simulink library "sm_robot_run_4legs_lib"  (R2025a)
settings: Solver=ode45  StartTime=0.0  StopTime=10.0  RelTol=1e-3
values from neighbouring files (symbols this model uses):
  N = 100    [Extr_Data_Cam_Roller_Curve.m]
  s = sin(q)    [Extr_Data_Cam_Roller_Curve.m]
undefined symbols (not defined in the file or in its folder): bw, d2r, Extr_Data_LinkEndHole, ground, J, joint_damping, k2, knee_torque, l1, l2, L_back, m1, m2, r2d, T_cg, t_th, t_w, th2, Trq_propulsive, u_th, u_w, X, Y, Z
libraries: sm_lib x25, nesl_utility x14, fl_lib x13, Contact_Forces_Lib x1, ee_lib x1
(part 1 of 2)
Description:
  | Copyright 2012-2025 The MathWorks, Inc.
settings Model: Creator=rhyde  LastModifiedBy=smiller
settings SolverCC: AlgebraicLoopSolver=TrustRegion
settings DataIOCC: SaveFormat=Array  SignalLoggingSaveFormat=ModelDataLogs  ReturnWorkspaceOutputs=off
settings OptimizationCC: BlockReduction=off  BooleanDataType=off  ReuseModelBlockBuffer=off  ExpressionDepthLimit=2147483647.0  LifeSpan=inf
settings DebuggingCC: SaveWithParameterizedLinksMsg=none  UnderspecifiedInitializationDetection=Classic  MergeDetectMultiDrivingBlocksExec=none  SignalResolutionControl=TryResolveAllWithWarning  UnconnectedInputMsg=warning  UnconnectedOutputMsg=warning  UnconnectedLineMsg=warning  StateNameClashWarn=warning  PregeneratedLibrarySubsystemCodeDiagnostic=none  SFUnexpectedBacktrackingDiag=warning  SFNoUnconditionalDefaultTransitionDiag=warning  SFExecutionAtInitializationDiag=none  ArithmeticOperatorsInVariantConditions=warning
settings HardwareCC: ProdBitPerPointer=32.0  ProdBitPerSizeT=32.0  ProdBitPerPtrDiffT=32.0  ProdLargestAtomicFloat=None  ProdIntDivRoundTo=Undefined  ProdEndianess=Unspecified  ProdWordSize=32.0  ProdHWDeviceType=32-bit Generic  TargetUnknown=on
settings ModelReferenceCC: EnableRefExpFcnMdlSchedulingChecks=on  PropagateSignalLabelsOutOfModel=off
settings SFSimCC: SimUseLocalCustomCode=off  CustomCodeUndefinedFunction=UseInterfaceOnly
settings RTWCC: RTWUseLocalCustomCode=off  GPUComputeCapability=3.5  DLArmComputeVersion=19.05
settings CodeAppCC: StateflowObjectComments=on
settings GRTTargetCC: TargetLangStandard=C89/C90 (ANSI)
settings ConfigComp: CovMetricSettings=dw  CovSaveCumulativeToWorkspaceVar=on  CovSaveSingleToWorkspaceVar=on  CovExternalEMLEnable=off

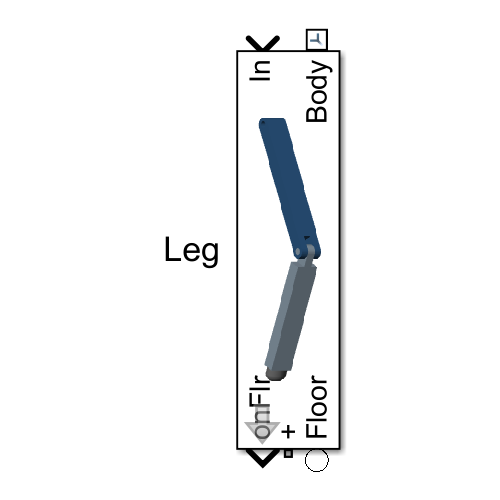
[thumbnail: Simulink's stored preview of the top-level diagram]
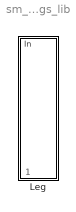
== system sm_robot_run_4legs_lib ==
  Leg : Subsystem  Tag=PublishSubsystemCustomStyle  mask{leg_type=Front Left, leg_width=0.1*l1, th1_0=d2r*u_th(find(t_th > 3*T_cg/4,1)), th2_0=-50*d2r+th2, th1_dot_0=-d2r*u_w(find(t_th > 3*T_cg/4,1)), x0=L_back, popup_contact_model=Planar}
      mask prompts: leg_type "Leg type"; leg_width "Leg width (m)"; th1_0 "Initial hip angle, th1_0"; th2_0 "Initial knee angle, th2_0"; th1_dot_0 "Initial hip angular velocity"; x0 "Current or last ground contact position, x0"; popup_contact_model "Contact Force Model"
      mask init:
      | if (leg_type == 1 || leg_type == 3)
      |     sideSign = -1;
      | else
      |     sideSign = 1;
      | end
      | 
      | if (popup_contact_model==1)
      |     set_param([gcb '/Contact Force Model'],'OverrideUsingVariant','Planar');
      | else
      |     set_param([gcb '/Contact Force Model'],'OverrideUsingVariant','SixDOF');
      | end
      mask TypeOptions leg_type: Front Left | Front Right | Rear Left | Rear Right
      mask TypeOptions popup_contact_model: Planar | Six DOF
      mask Display: image('sm_robot_run_leg_IMAGE.png')

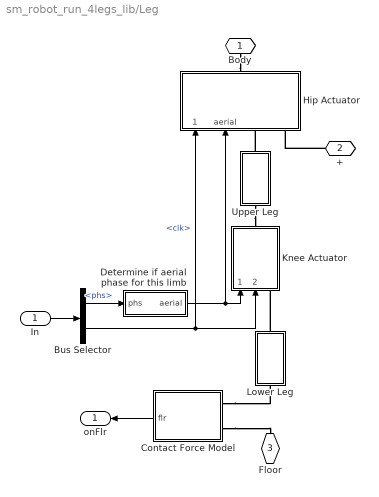
== system sm_robot_run_4legs_lib/Leg ==
  In : Inport
  Bus Selector : BusSelector  OutputSignals=phs,clk
  Contact Force Model : Subsystem  Variant=on  VariantControlMode=label  VariantControl=ThreeDim  LabelModeActiveChoice=Planar
      settings: AttributesFormatString=%<ActiveVariant>
      mask Display: disp(' ');
  Determine if aerial phase for this limb : Subsystem
  Hip Actuator : Subsystem
  Knee Actuator : Subsystem
  Lower Leg : Subsystem
  Upper Leg : Subsystem
  Body : PMIOPort  Side=Left
  + : PMIOPort  Port=2  Side=Right
  Floor : PMIOPort  Tag=PMCPort  Port=3  Side=Right
  onFlr : Outport  VectorParamsAs1DForOutWhenUnconnected=off
  wires:
  Contact Force Model/1("  flr") -> onFlr/1
  Bus Selector/2 -> Knee Actuator/2(t_aerial), Hip Actuator/1(t_aerial)  "<clk>"
  Determine if aerial phase for this limb/1(aerial) -> Knee Actuator/1(aerial), Hip Actuator/2(aerial)
  In/1 -> Bus Selector/1
  Bus Selector/1 -> Determine if aerial phase for this limb/1(phs)  "<phs>"
  connections:
  Body/RConn1 -- Hip Actuator/RConn1
  +/RConn1 -- Hip Actuator/LConn2
  Lower Leg/RConn1 -- Knee Actuator/LConn1
  Contact Force Model/LConn1 -- Lower Leg/LConn1
  Upper Leg/RConn1 -- Hip Actuator/LConn1
  Upper Leg/LConn1 -- Knee Actuator/RConn1
  Contact Force Model/LConn2 -- Floor/RConn1

== system sm_robot_run_4legs_lib/Leg/Contact Force Model ==
  Planar : Subsystem  VariantControl=Planar
  SixDOF : Subsystem  VariantControl=SixDOF
  " F " : PMIOPort  Side=Left
  " W " : PMIOPort  Port=2  Side=Left
  "  flr" : Outport  VectorParamsAs1DForOutWhenUnconnected=off

== system sm_robot_run_4legs_lib/Leg/Determine if aerial phase for this limb ==
  phs : Inport
  Aerial : Switch  Threshold=0.5  SaturateOnIntegerOverflow=off  InputSameDT=off
  "Front left or rear right leg airborne if phase is 1, 2, 3, 6, 7 or 8" : Fcn  Expr=(u(1)==1)+(u(1)==2)+(u(1)==3)+(u(1)==6)+(u(1)==7)+(u(1)==8)
  "Front right or rear left leg airborne if phase is 2, 3, 4, 5, 6 or 7" : Fcn  Expr=(u(1)==2)+(u(1)==3)+(u(1)==4)+(u(1)==5)+(u(1)==6)+(u(1)==7)
  Leg type is front right or rear left : Constant  Value=(leg_type==2)+(leg_type==3)
  aerial : Outport  VectorParamsAs1DForOutWhenUnconnected=off
  wires:
  Leg type is front right or rear left/1 -> Aerial/2
  "Front right or rear left leg airborne if phase is 2, 3, 4, 5, 6 or 7"/1 -> Aerial/1
  phs/1 -> "Front right or rear left leg airborne if phase is 2, 3, 4, 5, 6 or 7"/1, "Front left or rear right leg airborne if phase is 1, 2, 3, 6, 7 or 8"/1
  "Front left or rear right leg airborne if phase is 1, 2, 3, 6, 7 or 8"/1 -> Aerial/3
  Aerial/1 -> aerial/1

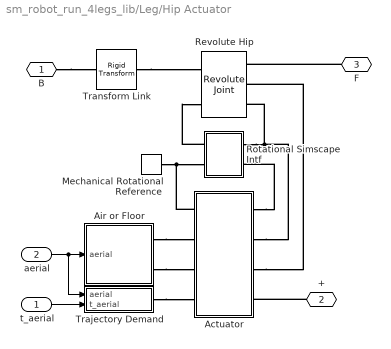
== system sm_robot_run_4legs_lib/Leg/Hip Actuator ==
  t_aerial : Inport
  aerial : Inport  Port=2
  Actuator : Subsystem
  Air or Floor : Subsystem
  Mechanical Rotational Reference : fl_lib/Mechanical/Rotational Elements/Mechanical Rotational Reference
  Revolute Hip : sm_lib/Joints/Revolute Joint  JointMode=Normal  CompositeWrenchDir=FollowerOnBase  CompositeWrenchFrame=BaseFrame  SenseConstraintForce=off  SenseConstraintTorque=off  SenseTotalForce=off  SenseTotalTorque=off  PositionTargetSpecify=on  PositionTargetPriority=High  PositionTargetValue=-th1_0  PositionTargetValueUnits=rad  VelocityTargetSpecify=on  VelocityTargetPriority=High  VelocityTargetValue=th1_dot_0  VelocityTargetValueUnits=rad/s  EquilibriumPosition=0  EquilibriumPositionUnits=deg  SpringStiffness=0  SpringStiffnessUnits=N*m/deg  DampingCoefficient=0  DampingCoefficientUnits=N*m/(deg/s)  LowerLimitSpecify=off  LowerLimitBound=-90  LowerLimitBoundUnits=deg  LowerLimitStiffness=1e4  LowerLimitStiffnessUnits=N*m/deg  LowerLimitDamping=10  LowerLimitDampingUnits=N*m/(deg/s)  LowerLimitTransitionRegionWidth=0.1  LowerLimitTransitionRegionWidthUnits=deg  UpperLimitSpecify=off  UpperLimitBound=90  UpperLimitBoundUnits=deg  UpperLimitStiffness=1e4  UpperLimitStiffnessUnits=N*m/deg  UpperLimitDamping=10  UpperLimitDampingUnits=N*m/(deg/s)  UpperLimitTransitionRegionWidth=0.1  UpperLimitTransitionRegionWidthUnits=deg  TorqueActuationMode=InputTorque  MotionActuationMode=ComputedMotion  SensePosition=on  SenseVelocity=on  SenseAcceleration=off  SenseTorqueForce=off  SenseLowerLimitTorqueForce=off  SenseUpperLimitTorqueForce=off
  Rotational Simscape Intf : Subsystem
  Trajectory Demand : Subsystem
  Transform Link : sm_lib/Frames and Transforms/Rigid Transform  RotationMethod=None  FollAlignAxisA=+X  BaseAlignAxisA=+Y  FollAlignAxisB=+Y  BaseAlignAxisB=+Z  RotationStandardAxis=+Z  RotationAngle=0.0  RotationAngleUnits=deg  RotationArbitraryAxis=[0 0 1]  RotationSequenceAxes=FollowerAxes  RotationSequence=XYX  RotationSequenceAngles=[0 0 0]  RotationSequenceAnglesUnits=deg  RotationMatrix=[1 0 0; 0 1 0; 0 0 1]  Quaternion=[1 0 0 0]  TranslationMethod=StandardAxis  TranslationCartesianOffset=[0 0 0]  TranslationCartesianOffsetUnits=m  TranslationStandardAxis=+Z  TranslationStandardOffset=leg_width*sideSign/2  TranslationStandardOffsetUnits=m  TranslationROffset=0  TranslationROffsetUnits=m  TranslationThetaOffset=0  TranslationThetaOffsetUnits=deg  TranslationZOffset=0  TranslationZOffsetUnits=m
  B : PMIOPort  Side=Left
  + : PMIOPort  Port=2  Side=Left
  F : PMIOPort  Port=3  Side=Right
  wires:
  aerial/1 -> Trajectory Demand/1(aerial), Air or Floor/1(aerial)
  t_aerial/1 -> Trajectory Demand/2(t_aerial)
  connections:
  Trajectory Demand/RConn1 -- Actuator/LConn4
  Mechanical Rotational Reference/LConn1 -- Actuator/LConn1 -- Rotational Simscape Intf/LConn2
  +/RConn1 -- Actuator/RConn4
  Transform Link/RConn1 -- Revolute Hip/LConn1
  F/RConn1 -- Revolute Hip/RConn1
  Actuator/RConn3 -- Revolute Hip/RConn2
  Rotational Simscape Intf/RConn1 -- Actuator/RConn2 -- Revolute Hip/RConn3
  Rotational Simscape Intf/LConn1 -- Revolute Hip/LConn2
  B/RConn1 -- Transform Link/LConn1
  Actuator/RConn1 -- Rotational Simscape Intf/RConn2
  Air or Floor/RConn2 -- Actuator/LConn3
  Air or Floor/RConn1 -- Actuator/LConn2

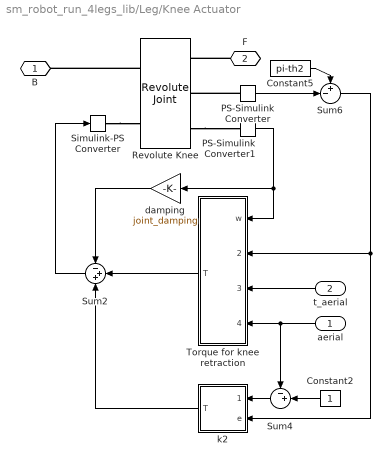
== system sm_robot_run_4legs_lib/Leg/Knee Actuator ==
  aerial : Inport
  t_aerial : Inport  Port=2
  Constant2 : Constant
  Constant5 : Constant  Value=pi-th2
  PS-Simulink Converter : nesl_utility/PS-Simulink Converter  PhysicalDomain=network_engine_domain  SubClassName=ps_output  LeftPortType=input  RightPortType=output  PseudoPeriodic=off  Frequencies=[]  VectorFormat=1-D array  Unit=rad  AffineConversion=off
  PS-Simulink Converter1 : nesl_utility/PS-Simulink Converter  PhysicalDomain=network_engine_domain  SubClassName=ps_output  LeftPortType=input  RightPortType=output  PseudoPeriodic=off  Frequencies=[]  VectorFormat=1-D array  Unit=rad/s  AffineConversion=off
  Revolute Knee : sm_lib/Joints/Revolute Joint  JointMode=Normal  CompositeWrenchDir=FollowerOnBase  CompositeWrenchFrame=BaseFrame  SenseConstraintForce=off  SenseConstraintTorque=off  SenseTotalForce=off  SenseTotalTorque=off  PositionTargetSpecify=on  PositionTargetPriority=High  PositionTargetValue=-th2_0+pi  PositionTargetValueUnits=rad  VelocityTargetSpecify=on  VelocityTargetPriority=High  VelocityTargetValue=0  VelocityTargetValueUnits=rad/s  EquilibriumPosition=0  EquilibriumPositionUnits=deg  SpringStiffness=0  SpringStiffnessUnits=N*m/deg  DampingCoefficient=0  DampingCoefficientUnits=N*m/(deg/s)  LowerLimitSpecify=off  LowerLimitBound=-90  LowerLimitBoundUnits=deg  LowerLimitStiffness=1e4  LowerLimitStiffnessUnits=N*m/deg  LowerLimitDamping=10  LowerLimitDampingUnits=N*m/(deg/s)  LowerLimitTransitionRegionWidth=0.1  LowerLimitTransitionRegionWidthUnits=deg  UpperLimitSpecify=off  UpperLimitBound=90  UpperLimitBoundUnits=deg  UpperLimitStiffness=1e4  UpperLimitStiffnessUnits=N*m/deg  UpperLimitDamping=10  UpperLimitDampingUnits=N*m/(deg/s)  UpperLimitTransitionRegionWidth=0.1  UpperLimitTransitionRegionWidthUnits=deg  TorqueActuationMode=InputTorque  MotionActuationMode=ComputedMotion  SensePosition=on  SenseVelocity=on  SenseAcceleration=off  SenseTorqueForce=off  SenseLowerLimitTorqueForce=off  SenseUpperLimitTorqueForce=off
  Simulink-PS Converter : nesl_utility/Simulink-PS Converter  PhysicalDomain=network_engine_domain  SubClassName=ps_input  LeftPortType=input  RightPortType=output  PseudoPeriodic=off  Frequencies=[]  NoiseDistribution=none  NoiseParameters=[]  Unit=1  AffineConversion=off  FilteringAndDerivatives=provide  SimscapeFilterOrder=1  InputFilterTimeConstant=0.005  UdotUserProvided=0
  Sum2 : Sum  Inputs=-++  InputSameDT=on  SaturateOnIntegerOverflow=on  OutDataTypeStr=Inherit: Same as first input
  Sum4 : Sum  Inputs=-+|  InputSameDT=on  SaturateOnIntegerOverflow=on  OutDataTypeStr=Inherit: Same as first input
  Sum6 : Sum  Inputs=+-|  InputSameDT=on  SaturateOnIntegerOverflow=on  OutDataTypeStr=Inherit: Same as first input
  Torque for knee retraction : Subsystem
  damping : Gain  Gain=joint_damping  SaturateOnIntegerOverflow=on  OutDataTypeStr=Inherit: Same as input  ParamDataTypeStr=Inherit: Same as input
  k2 : Subsystem
  B : PMIOPort  Side=Left
  F : PMIOPort  Port=2  Side=Right
  wires:
  Torque for knee retraction/1(T) -> Sum2/2
  k2/1(T) -> Sum2/3
  Constant2/1 -> Sum4/2
  Sum4/1 -> k2/1(Enable)
  aerial/1 -> Sum4/1, Torque for knee retraction/4(Enable)
  Sum6/1 -> k2/2(e), Torque for knee retraction/2(angle)
  damping/1 -> Sum2/1
  PS-Simulink Converter1/1 -> Torque for knee retraction/1(w), damping/1
  Sum2/1 -> Simulink-PS Converter/1
  t_aerial/1 -> Torque for knee retraction/3(t_aerial)
  PS-Simulink Converter/1 -> Sum6/2
  Constant5/1 -> Sum6/1
  connections:
  F/RConn1 -- Revolute Knee/RConn1
  PS-Simulink Converter/LConn1 -- Revolute Knee/RConn2
  Revolute Knee/RConn3 -- PS-Simulink Converter1/LConn1
  Simulink-PS Converter/RConn1 -- Revolute Knee/LConn2
  Revolute Knee/LConn1 -- B/RConn1

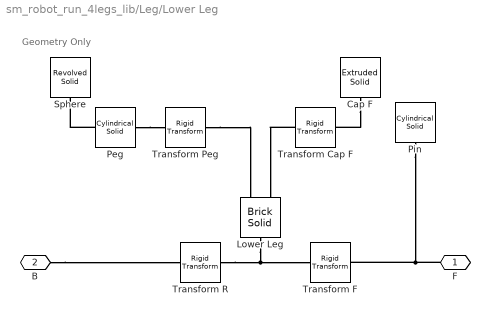
== system sm_robot_run_4legs_lib/Leg/Lower Leg ==
  note: Geometry Only
  Cap F : sm_lib/Body Elements/Extruded Solid  ExtrusionType=General  PolygonNumSides=3  PolygonOuterRadius=1  PolygonOuterRadiusUnits=m  ExportEntireGeometry=off  ExtrusionCrossSection=Extr_Data_LinkEndHole(l2*0.1,l1*0.025,0.05*l2)  ExtrusionCrossSectionUnits=m  ExportConvexHullGeometry=off  ExtrusionLength=l2*0.1/3  ExtrusionLengthUnits=m  InertiaType=CalculateFromGeometry  BasedOnType=Density  Density=0  DensityUnits=kg/m^3  Mass=1  MassUnits=kg  CenterOfMass=[0 0 0]  CenterOfMassUnits=m  MomentsOfInertia=[1 1 1]  MomentsOfInertiaUnits=kg*m^2  ProductsOfInertia=[1 1 1]  ProductsOfInertiaUnits=kg*m^2  GraphicType=FromGeometry  MarkerShape=Sphere  MarkerSize=10  GraphicVisPropType=SimpleVisualProperties  GraphicDiffuseColor=[164 184 200]/255  GraphicOpacity=1.0  GraphicSpecularColor=[0.5 0.5 0.5 1.0]  GraphicAmbientColor=[0.15 0.15 0.15 1.0]  GraphicEmissiveColor=[0.0 0.0 0.0 1.0]  GraphicShininess=75  DoExposeReferenceFrame=on  SerializedFrames=<Frames/>
  Lower Leg : sm_lib/Body Elements/Brick Solid  BrickDimensions=[0.1 0.8 0.1]*l2  BrickDimensionsUnits=m  ExportEntireGeometry=off  InertiaType=Custom  BasedOnType=Density  Density=1000  DensityUnits=kg/m^3  Mass=m2*l2  MassUnits=kg  CenterOfMass=[0 0 0]  CenterOfMassUnits=m  MomentsOfInertia=[1 1 1]*(1/12)*m2*l2*l2^2  MomentsOfInertiaUnits=kg*m^2  ProductsOfInertia=[1 1 1]*0  ProductsOfInertiaUnits=kg*m^2  GraphicType=FromGeometry  MarkerShape=Sphere  MarkerSize=10  GraphicVisPropType=SimpleVisualProperties  GraphicDiffuseColor=[164 184 200]/255  GraphicOpacity=1.0  GraphicSpecularColor=[0.5 0.5 0.5 1.0]  GraphicAmbientColor=[0.15 0.15 0.15 1.0]  GraphicEmissiveColor=[0.0 0.0 0.0 1.0]  GraphicShininess=75  DoExposeReferenceFrame=on  SerializedFrames=<Frames><Frame><Id>Frame1</Id><Value><Name>B</Name><Origin><Source>GeometricFeature</Source><FeatureName>-y surface</FeatureName></Origin><PrimaryAxis><DefinedDirection>+Z</DefinedDirection><Source>ReferenceFrame</Source><SourceDirection>+Z</SourceDirection><FeatureName></FeatureName></PrimaryAxis><SecondaryAxis><DefinedDirection>+X</DefinedDirection><Source>ReferenceFrame</Source><SourceDirection>+X</SourceDirection><FeatureName></FeatureName></SecondaryAxis></Value></Frame><Frame><Id>Frame2</Id><Value><Name>F</Name><Origin><Source>GeometricFeature</Source><FeatureName>+y surface</FeatureName></Origin><PrimaryAxis><DefinedDirection>+Z</DefinedDirection><Source>ReferenceFrame</Source><SourceDirection>+Z</SourceDirection><FeatureName></FeatureName></PrimaryAxis><SecondaryAxis><DefinedDirection>+X</DefinedDirection><Source>ReferenceFrame</Source><SourceDirection>+X</SourceDirection><FeatureName></FeatureName></SecondaryAxis></Value></Frame></Frames>
  Peg : sm_lib/Body Elements/Cylindrical Solid  CylinderRadius=0.05*l1  CylinderRadiusUnits=m  CylinderLength=0.05*l2  CylinderLengthUnits=m  ExportEntireGeometry=off  InertiaType=CalculateFromGeometry  BasedOnType=Density  Density=0  DensityUnits=kg/m^3  Mass=1  MassUnits=kg  CenterOfMass=[0 0 0]  CenterOfMassUnits=m  MomentsOfInertia=[1 1 1]  MomentsOfInertiaUnits=kg*m^2  ProductsOfInertia=[1 1 1]  ProductsOfInertiaUnits=kg*m^2  GraphicType=FromGeometry  MarkerShape=Sphere  MarkerSize=10  GraphicVisPropType=SimpleVisualProperties  GraphicDiffuseColor=[0.5 0.5 0.5]  GraphicOpacity=1.0  GraphicSpecularColor=[0.5 0.5 0.5 1.0]  GraphicAmbientColor=[0.15 0.15 0.15 1.0]  GraphicEmissiveColor=[0.0 0.0 0.0 1.0]  GraphicShininess=75  DoExposeReferenceFrame=off  SerializedFrames=<Frames><Frame><Id>Frame1</Id><Value><Name>B</Name><Origin><Source>GeometricFeature</Source><FeatureName>bottom surface</FeatureName></Origin><PrimaryAxis><DefinedDirection>+Z</DefinedDirection><Source>ReferenceFrame</Source><SourceDirection>+Z</SourceDirection><FeatureName></FeatureName></PrimaryAxis><SecondaryAxis><DefinedDirection>+X</DefinedDirection><Source>ReferenceFrame</Source><SourceDirection>+X</SourceDirection><FeatureName></FeatureName></SecondaryAxis></Value></Frame><Frame><Id>Frame2</Id><Value><Name>F</Name><Origin><Source>GeometricFeature</Source><FeatureName>top surface</FeatureName></Origin><PrimaryAxis><DefinedDirection>+Z</DefinedDirection><Source>ReferenceFrame</Source><SourceDirection>+Z</SourceDirection><FeatureName></FeatureName></PrimaryAxis><SecondaryAxis><DefinedDirection>+X</DefinedDirection><Source>ReferenceFrame</Source><SourceDirection>+X</SourceDirection><FeatureName></FeatureName></SecondaryAxis></Value></Frame></Frames>
  Pin : sm_lib/Body Elements/Cylindrical Solid  CylinderRadius=0.025*l1  CylinderRadiusUnits=m  CylinderLength=0.1*l2  CylinderLengthUnits=m  ExportEntireGeometry=off  InertiaType=CalculateFromGeometry  BasedOnType=Density  Density=0  DensityUnits=kg/m^3  Mass=1  MassUnits=kg  CenterOfMass=[0 0 0]  CenterOfMassUnits=m  MomentsOfInertia=[1 1 1]  MomentsOfInertiaUnits=kg*m^2  ProductsOfInertia=[1 1 1]  ProductsOfInertiaUnits=kg*m^2  GraphicType=FromGeometry  MarkerShape=Sphere  MarkerSize=10  GraphicVisPropType=SimpleVisualProperties  GraphicDiffuseColor=[164 184 200]/255  GraphicOpacity=1.0  GraphicSpecularColor=[0.5 0.5 0.5 1.0]  GraphicAmbientColor=[0.15 0.15 0.15 1.0]  GraphicEmissiveColor=[0.0 0.0 0.0 1.0]  GraphicShininess=75  DoExposeReferenceFrame=on  SerializedFrames=<Frames/>
  Sphere : sm_lib/Body Elements/Revolved Solid  RevolutionCrossSection=[sind(90:-1:0)' cosd(90:-1:0)']*l2*0.1/2  RevolutionCrossSectionUnits=m  RevolutionExtent=Full  RevolutionAngle=180  RevolutionAngleUnits=deg  ExportConvexHullGeometry=off  InertiaType=CalculateFromGeometry  BasedOnType=Density  Density=0  DensityUnits=kg/m^3  Mass=1  MassUnits=kg  CenterOfMass=[0 0 0]  CenterOfMassUnits=m  MomentsOfInertia=[1 1 1]  MomentsOfInertiaUnits=kg*m^2  ProductsOfInertia=[1 1 1]  ProductsOfInertiaUnits=kg*m^2  GraphicType=FromGeometry  MarkerShape=Sphere  MarkerSize=10  GraphicVisPropType=SimpleVisualProperties  GraphicDiffuseColor=[0.5 0.5 0.5]  GraphicOpacity=1.0  GraphicSpecularColor=[0.5 0.5 0.5 1.0]  GraphicAmbientColor=[0.15 0.15 0.15 1.0]  GraphicEmissiveColor=[0.0 0.0 0.0 1.0]  GraphicShininess=75  DoExposeReferenceFrame=on  SerializedFrames=<Frames/>
  Transform Cap F : sm_lib/Frames and Transforms/Rigid Transform  RotationMethod=StandardAxis  FollAlignAxisA=+X  BaseAlignAxisA=+Y  FollAlignAxisB=+Y  BaseAlignAxisB=+Z  RotationStandardAxis=+Z  RotationAngle=90  RotationAngleUnits=deg  RotationArbitraryAxis=[0 0 1]  RotationSequenceAxes=FollowerAxes  RotationSequence=XYX  RotationSequenceAngles=[0 0 0]  RotationSequenceAnglesUnits=deg  RotationMatrix=[1 0 0; 0 1 0; 0 0 1]  Quaternion=[1 0 0 0]  TranslationMethod=None  TranslationCartesianOffset=[0 0 0]  TranslationCartesianOffsetUnits=m  TranslationStandardAxis=+Z  TranslationStandardOffset=0  TranslationStandardOffsetUnits=m  TranslationROffset=0  TranslationROffsetUnits=m  TranslationThetaOffset=0  TranslationThetaOffsetUnits=deg  TranslationZOffset=0  TranslationZOffsetUnits=m
  Transform Peg : sm_lib/Frames and Transforms/Rigid Transform  RotationMethod=StandardAxis  FollAlignAxisA=+X  BaseAlignAxisA=+Y  FollAlignAxisB=+Y  BaseAlignAxisB=+Z  RotationStandardAxis=+X  RotationAngle=90  RotationAngleUnits=deg  RotationArbitraryAxis=[0 0 1]  RotationSequenceAxes=FollowerAxes  RotationSequence=XYX  RotationSequenceAngles=[0 0 0]  RotationSequenceAnglesUnits=deg  RotationMatrix=[1 0 0; 0 1 0; 0 0 1]  Quaternion=[1 0 0 0]  TranslationMethod=None  TranslationCartesianOffset=[0 0 0]  TranslationCartesianOffsetUnits=m  TranslationStandardAxis=+Z  TranslationStandardOffset=0  TranslationStandardOffsetUnits=m  TranslationROffset=0  TranslationROffsetUnits=m  TranslationThetaOffset=0  TranslationThetaOffsetUnits=deg  TranslationZOffset=0  TranslationZOffsetUnits=m
  Transform F : sm_lib/Frames and Transforms/Rigid Transform  RotationMethod=None  FollAlignAxisA=+X  BaseAlignAxisA=+Y  FollAlignAxisB=+Y  BaseAlignAxisB=+Z  RotationStandardAxis=+Z  RotationAngle=0.0  RotationAngleUnits=deg  RotationArbitraryAxis=[0 0 1]  RotationSequenceAxes=FollowerAxes  RotationSequence=XYX  RotationSequenceAngles=[0 0 0]  RotationSequenceAnglesUnits=deg  RotationMatrix=[1 0 0; 0 1 0; 0 0 1]  Quaternion=[1 0 0 0]  TranslationMethod=StandardAxis  TranslationCartesianOffset=[0 0 0]  TranslationCartesianOffsetUnits=m  TranslationStandardAxis=+Y  TranslationStandardOffset=l1/2  TranslationStandardOffsetUnits=m  TranslationROffset=0  TranslationROffsetUnits=m  TranslationThetaOffset=0  TranslationThetaOffsetUnits=deg  TranslationZOffset=0  TranslationZOffsetUnits=m
  Transform R : sm_lib/Frames and Transforms/Rigid Transform  RotationMethod=None  FollAlignAxisA=+X  BaseAlignAxisA=+Y  FollAlignAxisB=+Y  BaseAlignAxisB=+Z  RotationStandardAxis=+Z  RotationAngle=0.0  RotationAngleUnits=deg  RotationArbitraryAxis=[0 0 1]  RotationSequenceAxes=FollowerAxes  RotationSequence=XYX  RotationSequenceAngles=[0 0 0]  RotationSequenceAnglesUnits=deg  RotationMatrix=[1 0 0; 0 1 0; 0 0 1]  Quaternion=[1 0 0 0]  TranslationMethod=StandardAxis  TranslationCartesianOffset=[0 0 0]  TranslationCartesianOffsetUnits=m  TranslationStandardAxis=+Y  TranslationStandardOffset=l1/2  TranslationStandardOffsetUnits=m  TranslationROffset=0  TranslationROffsetUnits=m  TranslationThetaOffset=0  TranslationThetaOffsetUnits=deg  TranslationZOffset=0  TranslationZOffsetUnits=m
  F : PMIOPort  Side=Right
  B : PMIOPort  Port=2  Side=Left
  connections:
  B/RConn1 -- Transform R/LConn1
  F/RConn1 -- Pin/RConn1 -- Transform F/RConn1
  Lower Leg/RConn1 -- Transform R/RConn1 -- Transform F/LConn1
  Transform Cap F/LConn1 -- Lower Leg/LConn2
  Cap F/RConn1 -- Transform Cap F/RConn1
  Transform Peg/LConn1 -- Lower Leg/LConn1
  Peg/LConn1 -- Transform Peg/RConn1
  Peg/RConn1 -- Sphere/RConn1

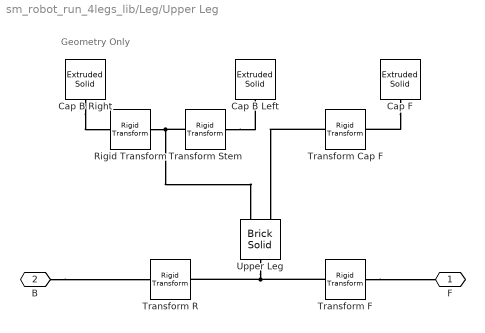
== system sm_robot_run_4legs_lib/Leg/Upper Leg ==
  note: Geometry Only
  Cap B Left : sm_lib/Body Elements/Extruded Solid  ExtrusionType=General  PolygonNumSides=3  PolygonOuterRadius=1  PolygonOuterRadiusUnits=m  ExportEntireGeometry=off  ExtrusionCrossSection=Extr_Data_LinkEndHole(l1*0.1,l1*0.025,0.05*l1)  ExtrusionCrossSectionUnits=m  ExportConvexHullGeometry=off  ExtrusionLength=l1*0.1/3  ExtrusionLengthUnits=m  InertiaType=CalculateFromGeometry  BasedOnType=Density  Density=0  DensityUnits=kg/m^3  Mass=1  MassUnits=kg  CenterOfMass=[0 0 0]  CenterOfMassUnits=m  MomentsOfInertia=[1 1 1]  MomentsOfInertiaUnits=kg*m^2  ProductsOfInertia=[1 1 1]  ProductsOfInertiaUnits=kg*m^2  GraphicType=FromGeometry  MarkerShape=Sphere  MarkerSize=10  GraphicVisPropType=SimpleVisualProperties  GraphicDiffuseColor=[0.2 0.4 0.6]  GraphicOpacity=1.0  GraphicSpecularColor=[0.5 0.5 0.5 1.0]  GraphicAmbientColor=[0.15 0.15 0.15 1.0]  GraphicEmissiveColor=[0.0 0.0 0.0 1.0]  GraphicShininess=75  DoExposeReferenceFrame=on  SerializedFrames=<Frames/>
  Cap B Right : sm_lib/Body Elements/Extruded Solid  ExtrusionType=General  PolygonNumSides=3  PolygonOuterRadius=1  PolygonOuterRadiusUnits=m  ExportEntireGeometry=off  ExtrusionCrossSection=Extr_Data_LinkEndHole(l1*0.1,l1*0.025,0.05*l1)  ExtrusionCrossSectionUnits=m  ExportConvexHullGeometry=off  ExtrusionLength=l1*0.1/3  ExtrusionLengthUnits=m  InertiaType=CalculateFromGeometry  BasedOnType=Density  Density=0  DensityUnits=kg/m^3  Mass=1  MassUnits=kg  CenterOfMass=[0 0 0]  CenterOfMassUnits=m  MomentsOfInertia=[1 1 1]  MomentsOfInertiaUnits=kg*m^2  ProductsOfInertia=[1 1 1]  ProductsOfInertiaUnits=kg*m^2  GraphicType=FromGeometry  MarkerShape=Sphere  MarkerSize=10  GraphicVisPropType=SimpleVisualProperties  GraphicDiffuseColor=[0.2 0.4 0.6]  GraphicOpacity=1.0  GraphicSpecularColor=[0.5 0.5 0.5 1.0]  GraphicAmbientColor=[0.15 0.15 0.15 1.0]  GraphicEmissiveColor=[0.0 0.0 0.0 1.0]  GraphicShininess=75  DoExposeReferenceFrame=on  SerializedFrames=<Frames/>
  Cap F : sm_lib/Body Elements/Extruded Solid  ExtrusionType=General  PolygonNumSides=3  PolygonOuterRadius=1  PolygonOuterRadiusUnits=m  ExportEntireGeometry=off  ExtrusionCrossSection=Extr_Data_LinkEndHole(l1*0.1,l1*0.025,0.05*l1)  ExtrusionCrossSectionUnits=m  ExportConvexHullGeometry=off  ExtrusionLength=l1*0.1  ExtrusionLengthUnits=m  InertiaType=CalculateFromGeometry  BasedOnType=Density  Density=0  DensityUnits=kg/m^3  Mass=1  MassUnits=kg  CenterOfMass=[0 0 0]  CenterOfMassUnits=m  MomentsOfInertia=[1 1 1]  MomentsOfInertiaUnits=kg*m^2  ProductsOfInertia=[1 1 1]  ProductsOfInertiaUnits=kg*m^2  GraphicType=FromGeometry  MarkerShape=Sphere  MarkerSize=10  GraphicVisPropType=SimpleVisualProperties  GraphicDiffuseColor=[0.2 0.4 0.6]  GraphicOpacity=1.0  GraphicSpecularColor=[0.5 0.5 0.5 1.0]  GraphicAmbientColor=[0.15 0.15 0.15 1.0]  GraphicEmissiveColor=[0.0 0.0 0.0 1.0]  GraphicShininess=75  DoExposeReferenceFrame=on  SerializedFrames=<Frames/>
  Rigid Transform : sm_lib/Frames and Transforms/Rigid Transform  RotationMethod=StandardAxis  FollAlignAxisA=+X  BaseAlignAxisA=+Y  FollAlignAxisB=+Y  BaseAlignAxisB=+Z  RotationStandardAxis=+Z  RotationAngle=-90  RotationAngleUnits=deg  RotationArbitraryAxis=[0 0 1]  RotationSequenceAxes=FollowerAxes  RotationSequence=XYX  RotationSequenceAngles=[0 0 0]  RotationSequenceAnglesUnits=deg  RotationMatrix=[1 0 0; 0 1 0; 0 0 1]  Quaternion=[1 0 0 0]  TranslationMethod=StandardAxis  TranslationCartesianOffset=[0 0 0]  TranslationCartesianOffsetUnits=m  TranslationStandardAxis=+Z  TranslationStandardOffset=0.1*l1/3  TranslationStandardOffsetUnits=m  TranslationROffset=0  TranslationROffsetUnits=m  TranslationThetaOffset=0  TranslationThetaOffsetUnits=deg  TranslationZOffset=0  TranslationZOffsetUnits=m
  Transform Cap F : sm_lib/Frames and Transforms/Rigid Transform  RotationMethod=StandardAxis  FollAlignAxisA=+X  BaseAlignAxisA=+Y  FollAlignAxisB=+Y  BaseAlignAxisB=+Z  RotationStandardAxis=+Z  RotationAngle=90  RotationAngleUnits=deg  RotationArbitraryAxis=[0 0 1]  RotationSequenceAxes=FollowerAxes  RotationSequence=XYX  RotationSequenceAngles=[0 0 0]  RotationSequenceAnglesUnits=deg  RotationMatrix=[1 0 0; 0 1 0; 0 0 1]  Quaternion=[1 0 0 0]  TranslationMethod=None  TranslationCartesianOffset=[0 0 0]  TranslationCartesianOffsetUnits=m  TranslationStandardAxis=+Z  TranslationStandardOffset=0  TranslationStandardOffsetUnits=m  TranslationROffset=0  TranslationROffsetUnits=m  TranslationThetaOffset=0  TranslationThetaOffsetUnits=deg  TranslationZOffset=0  TranslationZOffsetUnits=m
  Transform F : sm_lib/Frames and Transforms/Rigid Transform  RotationMethod=None  FollAlignAxisA=+X  BaseAlignAxisA=+Y  FollAlignAxisB=+Y  BaseAlignAxisB=+Z  RotationStandardAxis=+Z  RotationAngle=0.0  RotationAngleUnits=deg  RotationArbitraryAxis=[0 0 1]  RotationSequenceAxes=FollowerAxes  RotationSequence=XYX  RotationSequenceAngles=[0 0 0]  RotationSequenceAnglesUnits=deg  RotationMatrix=[1 0 0; 0 1 0; 0 0 1]  Quaternion=[1 0 0 0]  TranslationMethod=StandardAxis  TranslationCartesianOffset=[0 0 0]  TranslationCartesianOffsetUnits=m  TranslationStandardAxis=+Y  TranslationStandardOffset=l1/2  TranslationStandardOffsetUnits=m  TranslationROffset=0  TranslationROffsetUnits=m  TranslationThetaOffset=0  TranslationThetaOffsetUnits=deg  TranslationZOffset=0  TranslationZOffsetUnits=m
  Transform R : sm_lib/Frames and Transforms/Rigid Transform  RotationMethod=None  FollAlignAxisA=+X  BaseAlignAxisA=+Y  FollAlignAxisB=+Y  BaseAlignAxisB=+Z  RotationStandardAxis=+Z  RotationAngle=0.0  RotationAngleUnits=deg  RotationArbitraryAxis=[0 0 1]  RotationSequenceAxes=FollowerAxes  RotationSequence=XYX  RotationSequenceAngles=[0 0 0]  RotationSequenceAnglesUnits=deg  RotationMatrix=[1 0 0; 0 1 0; 0 0 1]  Quaternion=[1 0 0 0]  TranslationMethod=StandardAxis  TranslationCartesianOffset=[0 0 0]  TranslationCartesianOffsetUnits=m  TranslationStandardAxis=+Y  TranslationStandardOffset=l1/2  TranslationStandardOffsetUnits=m  TranslationROffset=0  TranslationROffsetUnits=m  TranslationThetaOffset=0  TranslationThetaOffsetUnits=deg  TranslationZOffset=0  TranslationZOffsetUnits=m
  "Transform Stem " : sm_lib/Frames and Transforms/Rigid Transform  RotationMethod=StandardAxis  FollAlignAxisA=+X  BaseAlignAxisA=+Y  FollAlignAxisB=+Y  BaseAlignAxisB=+Z  RotationStandardAxis=+Z  RotationAngle=-90  RotationAngleUnits=deg  RotationArbitraryAxis=[0 0 1]  RotationSequenceAxes=FollowerAxes  RotationSequence=XYX  RotationSequenceAngles=[0 0 0]  RotationSequenceAnglesUnits=deg  RotationMatrix=[1 0 0; 0 1 0; 0 0 1]  Quaternion=[1 0 0 0]  TranslationMethod=StandardAxis  TranslationCartesianOffset=[0 0 0]  TranslationCartesianOffsetUnits=m  TranslationStandardAxis=+Z  TranslationStandardOffset=-0.1*l1/3  TranslationStandardOffsetUnits=m  TranslationROffset=0  TranslationROffsetUnits=m  TranslationThetaOffset=0  TranslationThetaOffsetUnits=deg  TranslationZOffset=0  TranslationZOffsetUnits=m
  Upper Leg : sm_lib/Body Elements/Brick Solid  BrickDimensions=[0.1 0.8 0.1]*l1  BrickDimensionsUnits=m  ExportEntireGeometry=off  InertiaType=Custom  BasedOnType=Density  Density=1000  DensityUnits=kg/m^3  Mass=m1*l1  MassUnits=kg  CenterOfMass=[0 0 0]  CenterOfMassUnits=m  MomentsOfInertia=[1 1 1]*(1/12)*m1*l1*l1^2  MomentsOfInertiaUnits=kg*m^2  ProductsOfInertia=[1 1 1]*0  ProductsOfInertiaUnits=kg*m^2  GraphicType=FromGeometry  MarkerShape=Sphere  MarkerSize=10  GraphicVisPropType=SimpleVisualProperties  GraphicDiffuseColor=[0.2 0.4 0.6]  GraphicOpacity=1.0  GraphicSpecularColor=[0.5 0.5 0.5 1.0]  GraphicAmbientColor=[0.15 0.15 0.15 1.0]  GraphicEmissiveColor=[0.0 0.0 0.0 1.0]  GraphicShininess=75  DoExposeReferenceFrame=on  SerializedFrames=<Frames><Frame><Id>Frame1</Id><Value><Name>B</Name><Origin><Source>GeometricFeature</Source><FeatureName>-y surface</FeatureName></Origin><PrimaryAxis><DefinedDirection>+Z</DefinedDirection><Source>ReferenceFrame</Source><SourceDirection>+Z</SourceDirection><FeatureName></FeatureName></PrimaryAxis><SecondaryAxis><DefinedDirection>+X</DefinedDirection><Source>ReferenceFrame</Source><SourceDirection>+X</SourceDirection><FeatureName></FeatureName></SecondaryAxis></Value></Frame><Frame><Id>Frame2</Id><Value><Name>F</Name><Origin><Source>GeometricFeature</Source><FeatureName>+y surface</FeatureName></Origin><PrimaryAxis><DefinedDirection>+Z</DefinedDirection><Source>ReferenceFrame</Source><SourceDirection>+Z</SourceDirection><FeatureName></FeatureName></PrimaryAxis><SecondaryAxis><DefinedDirection>+X</DefinedDirection><Source>ReferenceFrame</Source><SourceDirection>+X</SourceDirection><FeatureName></FeatureName></SecondaryAxis></Value></Frame></Frames>
  F : PMIOPort  Side=Right
  B : PMIOPort  Port=2  Side=Left
  connections:
  B/RConn1 -- Transform R/LConn1
  Transform F/RConn1 -- F/RConn1
  Upper Leg/RConn1 -- Transform R/RConn1 -- Transform F/LConn1
  Cap B Right/RConn1 -- Rigid Transform/RConn1
  Cap F/RConn1 -- Transform Cap F/RConn1
  Rigid Transform/LConn1 -- "Transform Stem "/LConn1 -- Upper Leg/LConn1
  "Transform Stem "/RConn1 -- Cap B Left/RConn1
  Transform Cap F/LConn1 -- Upper Leg/LConn2

== system sm_robot_run_4legs_lib/Leg/Contact Force Model/Planar ==
  External Force and Torque : sm_lib/Forces and Torques/External Force and Torque  EnableForceX=off  EnableForceY=off  EnableForceZ=off  EnableForce=on  ForceResolutionFrame=World  EnableTorqueX=off  EnableTorqueY=off  EnableTorqueZ=off  EnableTorque=off  TorqueResolutionFrame=AttachedFrame
  Force Law : Subsystem
  Signals : Subsystem
  Simulink-PS Converter : nesl_utility/Simulink-PS Converter  PhysicalDomain=network_engine_domain  SubClassName=ps_input  LeftPortType=input  RightPortType=output  PseudoPeriodic=off  Frequencies=[]  NoiseDistribution=none  NoiseParameters=[]  Unit=1  AffineConversion=off  FilteringAndDerivatives=provide  SimscapeFilterOrder=1  InputFilterTimeConstant=0.005  UdotUserProvided=0
  Transform Sensor : sm_lib/Frames and Transforms/Transform Sensor  MeasurementFrame=World  RotationSequence=XYX  SenseAngle=off  SenseAxis=off  SenseQ=off  SenseR=off  SenseRotationSequence=off  SenseOmegaX=off  SenseOmegaY=off  SenseOmegaZ=off  SenseOmega=off  SenseQDot=off  SenseRDot=off  SenseRotationSequenceDot=off  SenseAlphaX=off  SenseAlphaY=off  SenseAlphaZ=off  SenseAlpha=off  SenseQDDot=off  SenseRDDot=off  SenseX=on  SenseY=on  SenseZ=on  SenseXYZ=off  SenseRad=off  SenseAzim=off  SenseDist=off  SenseInc=off  SenseXDot=on  SenseYDot=on  SenseZDot=on  SenseXYZDot=off  SenseRadDot=off  SenseAzimDot=off  SenseDistDot=off  SenseIncDot=off  SenseXDDot=off  SenseYDDot=off  SenseZDDot=off  SenseXYZDDot=off  SenseRadDDot=off  SenseAzimDDot=off  SenseDistDDot=off  SenseIncDDot=off
  F : PMIOPort  Side=Left
  W : PMIOPort  Port=2  Side=Left
  " flr" : Outport  VectorParamsAs1DForOutWhenUnconnected=off
  wires:
  Signals/2(v) -> Force Law/2(vel)
  Signals/1(p) -> Force Law/1(pos)
  Force Law/2(force) -> Simulink-PS Converter/1  "Force (N)"
  Force Law/1(on_floor) -> " flr"/1  "Foot on floor"
  connections:
  Simulink-PS Converter/RConn1 -- External Force and Torque/LConn1
  Transform Sensor/RConn5 -- Signals/LConn4
  Signals/LConn1 -- Transform Sensor/RConn2
  Signals/LConn3 -- Transform Sensor/RConn4
  W/RConn1 -- Transform Sensor/LConn1
  Signals/LConn2 -- Transform Sensor/RConn3
  Transform Sensor/RConn6 -- Signals/LConn5
  Transform Sensor/RConn7 -- Signals/LConn6
  Transform Sensor/RConn1 -- F/RConn1 -- External Force and Torque/RConn1

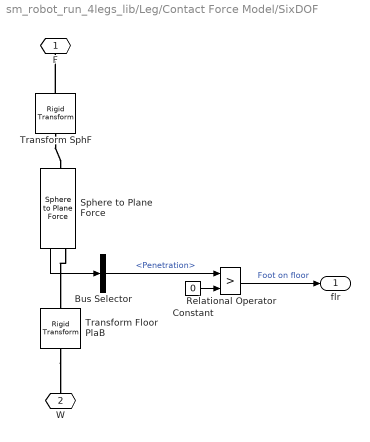
== system sm_robot_run_4legs_lib/Leg/Contact Force Model/SixDOF ==
  Bus Selector : BusSelector  OutputSignals=Penetration
  Constant : Constant  Value=0
  Relational Operator : RelationalOperator  Operator=>  OutDataTypeStr=boolean  InputSameDT=off
  Sphere to Plane Force : Contact_Forces_Lib/3D/Sphere to Plane Force  sphere_rad=0.1*l2/2  plane_lenx=100  plane_leny=100  plane_depth=0.05-l2*0.1/2*(1-sind(90-(-th2_0+pi)*180/pi-(-th1_0)*180/pi))  force_law=Linear  k_contact=ground.stiffness  b_contact=ground.damping  pen_full_damp_F=1e-4  pen_exponent=1  custom_param_1=1  custom_param_2=1  friction_law=Stick-Slip Continuous  mu_kinetic=0.88  mu_static=0.9  v_thr=0.001  vis_on=off  vis_opc_en=0  vis_len_plaBz=0.005  vis_clr=[0.9 0.2 0.2]  vis_opc=0.7
  Transform Floor PlaB : sm_lib/Frames and Transforms/Rigid Transform  RotationMethod=StandardAxis  FollAlignAxisA=+X  BaseAlignAxisA=+Y  FollAlignAxisB=+Y  BaseAlignAxisB=+Z  RotationStandardAxis=+X  RotationAngle=-90  RotationAngleUnits=deg  RotationArbitraryAxis=[0 0 1]  RotationSequenceAxes=FollowerAxes  RotationSequence=XYX  RotationSequenceAngles=[0 0 0]  RotationSequenceAnglesUnits=deg  RotationMatrix=[1 0 0; 0 1 0; 0 0 1]  Quaternion=[1 0 0 0]  TranslationMethod=StandardAxis  TranslationCartesianOffset=[0 0 0]  TranslationCartesianOffsetUnits=m  TranslationStandardAxis=-Y  TranslationStandardOffset=0.05  TranslationStandardOffsetUnits=m  TranslationROffset=0  TranslationROffsetUnits=m  TranslationThetaOffset=0  TranslationThetaOffsetUnits=deg  TranslationZOffset=0  TranslationZOffsetUnits=m
  Transform SphF : sm_lib/Frames and Transforms/Rigid Transform  RotationMethod=None  FollAlignAxisA=+X  BaseAlignAxisA=+Y  FollAlignAxisB=+Y  BaseAlignAxisB=+Z  RotationStandardAxis=+X  RotationAngle=-90  RotationAngleUnits=deg  RotationArbitraryAxis=[0 0 1]  RotationSequenceAxes=FollowerAxes  RotationSequence=XYX  RotationSequenceAngles=[0 0 0]  RotationSequenceAnglesUnits=deg  RotationMatrix=[1 0 0; 0 1 0; 0 0 1]  Quaternion=[1 0 0 0]  TranslationMethod=StandardAxis  TranslationCartesianOffset=[0 0 0]  TranslationCartesianOffsetUnits=m  TranslationStandardAxis=+Y  TranslationStandardOffset=0.1*l2/2  TranslationStandardOffsetUnits=m  TranslationROffset=0  TranslationROffsetUnits=m  TranslationThetaOffset=0  TranslationThetaOffsetUnits=deg  TranslationZOffset=0  TranslationZOffsetUnits=m
  F : PMIOPort  Side=Left
  W : PMIOPort  Port=2  Side=Left
  " flr" : Outport  VectorParamsAs1DForOutWhenUnconnected=off
  wires:
  Relational Operator/1 -> " flr"/1  "Foot on floor"
  Bus Selector/1 -> Relational Operator/1  "<Penetration>"
  Sphere to Plane Force/1 -> Bus Selector/1
  Constant/1 -> Relational Operator/2
  connections:
  Sphere to Plane Force/RConn1 -- Transform Floor PlaB/RConn1
  Transform SphF/RConn1 -- Sphere to Plane Force/LConn1
  Transform Floor PlaB/LConn1 -- W/RConn1
  Transform SphF/LConn1 -- F/RConn1

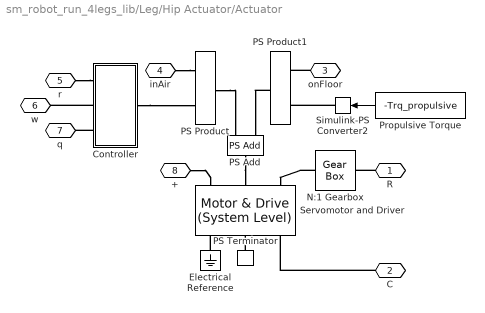
== system sm_robot_run_4legs_lib/Leg/Hip Actuator/Actuator ==
  Controller : Subsystem
  Electrical Reference : fl_lib/Electrical/Electrical Elements/Electrical Reference
  N:1 Gearbox : fl_lib/Mechanical/Mechanisms/Gear Box  ratio=-N  t_in_specify=off  t_in_priority=None  t_in=0 N*m  t_in_nominal_specify=off  t_in_nominal_value=1  t_in_nominal_unit=N*m  t_out_specify=off  t_out_priority=None  t_out=0 N*m  t_out_nominal_specify=off  t_out_nominal_value=1  t_out_nominal_unit=N*m
  PS Add : fl_lib/Physical Signals/Functions/PS Add
  PS Product : fl_lib/Physical Signals/Functions/PS Product
  PS Product1 : fl_lib/Physical Signals/Functions/PS Product
  PS Terminator : fl_lib/Physical Signals/Sinks/PS Terminator
  Propulsive Torque : Constant  Value=-Trq_propulsive
  Servomotor and Driver : ee_lib/Electromechanical/Motor & Drive (System Level)  torque_speed_param=1  overtorque_param=ee.enum.electromech.overtorque.no  T_t="[  0.13 0.115 0.1 0 ]*5 N*m"  T_t_intermittent=[.36, .32, .28, 0] N*m  T_t_2D=[.09, .09, .09; .08, .08, .08; .07, .07, .07; 0, 0, 0] N*m  T_t_intermittent_2D=[.36, .36, .36; .32, .32, .32; .28, .28, .28; 0, 0, 0] N*m  w_t="[  0 2e+03 4e+03 4.1e3] rpm"  vdc_t=[6, 12, 24] V  torque_max=0.1 N*m  power_max=30 W  torque_max_intermittent=0.4 N*m  power_max_intermittent=120 W  time_overtorque=30 s  time_recover=60 s  Tc=0.01 s  EnableSwitch=simscape.enum.onoff.off  losses_param=1  eff=100  w_eff=3.75e+3 rpm  T_eff=0.08 N*m  Piron=0 W  Pbase=0 W  w_eff_vec=[-8000 -4000 0 4000 8000] rpm  T_eff_vec=[0 0.03 0.06 0.09] N*m  v_eff_vec=[100, 250, 400] V  losses_mat=[1.49 1.67 2.21 3.10; 0.42 0.69 1.14 2.03; 0.06 0.24 0.78 1.68; 0.42 0.69 1.14 2.03; 1.49 1.67 2.21 3.10] W  efficiency_mat=[95 95 95 95; 95 95 95 95; 95 95 95 95; 95 95 95 95; 95 95 95 95]  losses_mat_3D=ones(5, 4, 3) W  efficiency_mat_3D=95 * ones(5, 4, 3)  Res=0.1 Ohm  J=0 g*cm^2  lam=0 N*m/(rad/s)  speed0=th1_dot_0*N rad/s  faulted_specify=off  faulted_priority=None  faulted=0  faulted_nominal_specify=off  faulted_nominal_value=1  faulted_nominal_unit=1  isSwitchedOff_specify=off  isSwitchedOff_priority=None  isSwitchedOff=0  isSwitchedOff_nominal_specify=off  isSwitchedOff_nominal_value=1  isSwitchedOff_nominal_unit=1  torqueLimitContinuous_specify=off  torqueLimitContinuous_priority=None  torqueLimitContinuous=0 N*m  torqueLimitContinuous_nominal_specify=off  torqueLimitContinuous_nominal_value=1  torqueLimitContinuous_nominal_unit=N*m  alpha=3.93e-3 1/K  Tmeas=25 degC  Tmeas2=125 degC  losses_mat_T2=[1.49, 1.74, 2.49, 3.74; .42, .67, 1.42, 2.67; .06, .31, 1.06, 2.31; .42, .67, 1.42, 2.67; 1.49, 1.74, 2.49, 3.74] W  efficiency_mat_T2=[95, 95, 95, 95; 95, 95, 95, 95; 95, 95, 95, 95; 95, 95, 95, 95; 95, 95, 95, 95]  losses_mat_3D_T2=ones(5, 4, 3) W  efficiency_mat_3D_T2=95 * ones(5, 4, 3)  thermal_mass=100 J/K  initial_temperature=25 degC
  Simulink-PS Converter2 : nesl_utility/Simulink-PS Converter  PhysicalDomain=network_engine_domain  SubClassName=ps_input  LeftPortType=input  RightPortType=output  PseudoPeriodic=off  Frequencies=[]  NoiseDistribution=none  NoiseParameters=[]  Unit=N*m  AffineConversion=off  FilteringAndDerivatives=zero  SimscapeFilterOrder=1  InputFilterTimeConstant=0.005  UdotUserProvided=0
  R : PMIOPort  Side=Right
  C : PMIOPort  Port=2  Side=Left
  onFloor : PMIOPort  Port=3  Side=Left
  inAir : PMIOPort  Port=4  Side=Left
  r : PMIOPort  Port=5  Side=Left
  w : PMIOPort  Port=6  Side=Right
  q : PMIOPort  Port=7  Side=Right
  + : PMIOPort  Port=8  Side=Right
  wires:
  Propulsive Torque/1 -> Simulink-PS Converter2/1
  connections:
  inAir/RConn1 -- PS Product/LConn2
  PS Terminator/LConn1 -- Servomotor and Driver/RConn2
  N:1 Gearbox/LConn1 -- Servomotor and Driver/LConn3
  R/RConn1 -- N:1 Gearbox/RConn1
  C/RConn1 -- Servomotor and Driver/RConn3
  Electrical Reference/LConn1 -- Servomotor and Driver/RConn1
  +/RConn1 -- Servomotor and Driver/LConn1
  Controller/RConn1 -- PS Product/LConn1
  r/RConn1 -- Controller/LConn1
  Controller/LConn3 -- q/RConn1
  Controller/LConn2 -- w/RConn1
  PS Add/RConn1 -- Servomotor and Driver/LConn2
  PS Product/RConn1 -- PS Add/LConn1
  onFloor/RConn1 -- PS Product1/LConn1
  PS Product1/RConn1 -- PS Add/LConn2
  Simulink-PS Converter2/RConn1 -- PS Product1/LConn2

== system sm_robot_run_4legs_lib/Leg/Hip Actuator/Air or Floor ==
  aerial : Inport
  Data Type Conversion : DataTypeConversion  OutDataTypeStr=double  SaturateOnIntegerOverflow=off  RndMeth=Floor
  On ground : Fcn  Expr=1-u
  Simulink-PS Converter : nesl_utility/Simulink-PS Converter  PhysicalDomain=network_engine_domain  SubClassName=ps_input  LeftPortType=input  RightPortType=output  PseudoPeriodic=off  Frequencies=[]  NoiseDistribution=none  NoiseParameters=[]  Unit=1  AffineConversion=off  FilteringAndDerivatives=zero  SimscapeFilterOrder=1  InputFilterTimeConstant=0.005  UdotUserProvided=0
  Simulink-PS Converter1 : nesl_utility/Simulink-PS Converter  PhysicalDomain=network_engine_domain  SubClassName=ps_input  LeftPortType=input  RightPortType=output  PseudoPeriodic=off  Frequencies=[]  NoiseDistribution=none  NoiseParameters=[]  Unit=1  AffineConversion=off  FilteringAndDerivatives=zero  SimscapeFilterOrder=1  InputFilterTimeConstant=0.005  UdotUserProvided=0
  onFloor : PMIOPort  Side=Right
  inAir : PMIOPort  Port=2  Side=Right
  wires:
  Data Type Conversion/1 -> On ground/1, Simulink-PS Converter/1
  On ground/1 -> Simulink-PS Converter1/1
  aerial/1 -> Data Type Conversion/1
  connections:
  Simulink-PS Converter/RConn1 -- inAir/RConn1
  Simulink-PS Converter1/RConn1 -- onFloor/RConn1

== system sm_robot_run_4legs_lib/Leg/Hip Actuator/Rotational Simscape Intf ==
  Angular Velocity Source : fl_lib/Mechanical/Mechanical Sources/Ideal Angular Velocity Source
  Torque Sensor : fl_lib/Mechanical/Mechanical Sensors/Ideal Torque Sensor
  w : PMIOPort  Side=Right
  t : PMIOPort  Port=2  Side=Left
  R : PMIOPort  Port=3  Side=Right
  C : PMIOPort  Port=4  Side=Left
  connections:
  Torque Sensor/RConn1 -- C/RConn1
  R/RConn1 -- Angular Velocity Source/LConn1
  Torque Sensor/LConn1 -- Angular Velocity Source/RConn2
  t/RConn1 -- Torque Sensor/RConn2
  w/RConn1 -- Angular Velocity Source/RConn1

== system sm_robot_run_4legs_lib/Leg/Hip Actuator/Trajectory Demand ==
  aerial : Inport
  t_aerial : Inport  Port=2
  Enabled Subsystem : Subsystem  TreatAsAtomicUnit=on
  Gain : Gain  Gain=d2r
  Simulink-PS Converter : nesl_utility/Simulink-PS Converter  PhysicalDomain=network_engine_domain  SubClassName=ps_input  LeftPortType=input  RightPortType=output  PseudoPeriodic=off  Frequencies=[]  NoiseDistribution=none  NoiseParameters=[]  Unit=rad  AffineConversion=off  FilteringAndDerivatives=zero  SimscapeFilterOrder=1  InputFilterTimeConstant=0.005  UdotUserProvided=0
  Terminator : Terminator
  Terminator1 : Terminator
  r : PMIOPort  Side=Right
  wires:
  Gain/1 -> Simulink-PS Converter/1
  aerial/1 -> Enabled Subsystem/Enable
  Enabled Subsystem/1(r) -> Gain/1
  t_aerial/1 -> Enabled Subsystem/1(t_aerial)
  Enabled Subsystem/2(angle) -> Terminator/1
  Enabled Subsystem/3(angle_dot) -> Terminator1/1
  connections:
  r/RConn1 -- Simulink-PS Converter/RConn1

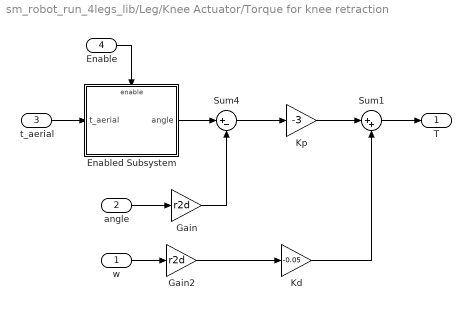
== system sm_robot_run_4legs_lib/Leg/Knee Actuator/Torque for knee retraction ==
  w : Inport
  angle : Inport  Port=2
  t_aerial : Inport  Port=3
  Enable : Inport  Port=4
  Enabled Subsystem : Subsystem  TreatAsAtomicUnit=on
  Gain : Gain  Gain=r2d
  Gain2 : Gain  Gain=r2d
  Kd : Gain  Gain=-0.05
  Kp : Gain  Gain=-3
  Sum1 : Sum  Inputs=|++  InputSameDT=on  SaturateOnIntegerOverflow=on  OutDataTypeStr=Inherit: Same as first input
  Sum4 : Sum  Inputs=|+-  InputSameDT=on  SaturateOnIntegerOverflow=on  OutDataTypeStr=Inherit: Same as first input
  T : Outport  VectorParamsAs1DForOutWhenUnconnected=off
  wires:
  Kd/1 -> Sum1/2
  Sum1/1 -> T/1
  Kp/1 -> Sum1/1
  Gain2/1 -> Kd/1
  w/1 -> Gain2/1
  Enabled Subsystem/1(angle) -> Sum4/1
  Gain/1 -> Sum4/2
  Sum4/1 -> Kp/1
  angle/1 -> Gain/1
  Enable/1 -> Enabled Subsystem/Enable
  t_aerial/1 -> Enabled Subsystem/1(t_aerial)

== system sm_robot_run_4legs_lib/Leg/Knee Actuator/k2 ==
  Enable : Inport
  e : Inport  Port=2
  Product : Product  RndMeth=Zero
  spring k2 : Gain  Gain=k2  SaturateOnIntegerOverflow=on  OutDataTypeStr=Inherit: Same as input  ParamDataTypeStr=Inherit: Same as input
  T : Outport  VectorParamsAs1DForOutWhenUnconnected=off
  wires:
  Enable/1 -> Product/1
  spring k2/1 -> Product/2
  Product/1 -> T/1
  e/1 -> spring k2/1

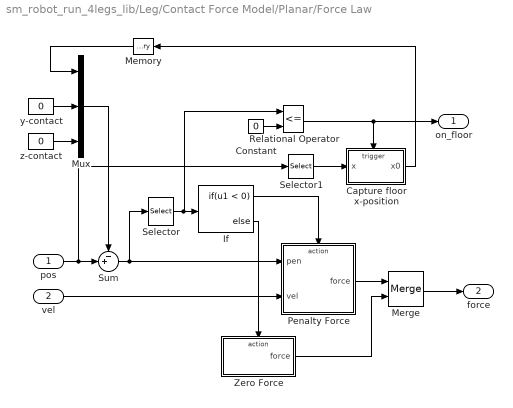
== system sm_robot_run_4legs_lib/Leg/Contact Force Model/Planar/Force Law ==
  pos : Inport
  vel : Inport  Port=2
  Capture floor x-position : Subsystem  TreatAsAtomicUnit=on
  Constant : Constant  Value=0
  If : If  IfExpression=u1 < 0
  Memory : Memory  InitialCondition=x0
  Merge : Merge  InitialOutput=0  InputPortOffsets=0
  Mux : Mux  Inputs=3
  Penalty Force : Subsystem  TreatAsAtomicUnit=on
  Relational Operator : RelationalOperator  Operator=<=  OutDataTypeStr=boolean  InputSameDT=off
  Selector : Selector  InputPortWidth=3  IndexOptions=Index vector (dialog)  Indices=2  OutputSizes=1
  Selector1 : Selector  InputPortWidth=3  IndexOptions=Index vector (dialog)  Indices=1  OutputSizes=1
  Sum : Sum  Inputs=-+|
  Zero Force : Subsystem  TreatAsAtomicUnit=on
  y-contact : Constant  Value=0
  z-contact : Constant  Value=0
  on_floor : Outport  VectorParamsAs1DForOutWhenUnconnected=off
  force : Outport  Port=2  VectorParamsAs1DForOutWhenUnconnected=off
  wires:
  vel/1 -> Penalty Force/2(vel)
  If/2 -> Zero Force/Action
  Penalty Force/1(force) -> Merge/1
  Zero Force/1(force) -> Merge/2
  If/1 -> Penalty Force/Action
  Selector/1 -> If/1, Relational Operator/1
  Constant/1 -> Relational Operator/2
  Relational Operator/1 -> Capture floor x-position/Trigger, on_floor/1
  Selector1/1 -> Capture floor x-position/1(x)
  z-contact/1 -> Mux/3
  y-contact/1 -> Mux/2
  Capture floor x-position/1(x0) -> Memory/1
  pos/1 -> Sum/2, Selector1/1
  Sum/1 -> Penalty Force/1(pen), Selector/1
  Mux/1 -> Sum/1
  Memory/1 -> Mux/1
  Merge/1 -> force/1

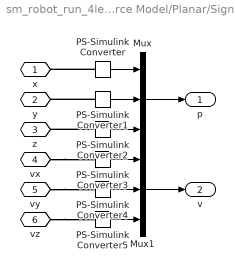
== system sm_robot_run_4legs_lib/Leg/Contact Force Model/Planar/Signals ==
  Mux : Mux  Inputs=3
  Mux1 : Mux  Inputs=3
  PS-Simulink Converter{,1..5} (6 alike) : nesl_utility/PS-Simulink Converter  PhysicalDomain=network_engine_domain  SubClassName=ps_output  LeftPortType=input  RightPortType=output  PseudoPeriodic=off  Frequencies=[]  VectorFormat=1-D array  Unit=1  AffineConversion=off
  x : PMIOPort  Side=Left
  y : PMIOPort  Port=2  Side=Left
  z : PMIOPort  Port=3  Side=Left
  vx : PMIOPort  Port=4  Side=Left
  vy : PMIOPort  Port=5  Side=Left
  vz : PMIOPort  Port=6  Side=Left
  p : Outport  VectorParamsAs1DForOutWhenUnconnected=off
  v : Outport  Port=2  VectorParamsAs1DForOutWhenUnconnected=off
  wires:
  Mux/1 -> p/1
  PS-Simulink Converter1/1 -> Mux/2
  PS-Simulink Converter2/1 -> Mux/3
  PS-Simulink Converter/1 -> Mux/1
  PS-Simulink Converter4/1 -> Mux1/2
  PS-Simulink Converter5/1 -> Mux1/3
  Mux1/1 -> v/1
  PS-Simulink Converter3/1 -> Mux1/1
  connections:
  PS-Simulink Converter1/LConn1 -- y/RConn1
  PS-Simulink Converter/LConn1 -- x/RConn1
  vz/RConn1 -- PS-Simulink Converter5/LConn1
  vx/RConn1 -- PS-Simulink Converter3/LConn1
  vy/RConn1 -- PS-Simulink Converter4/LConn1
  PS-Simulink Converter2/LConn1 -- z/RConn1

== system sm_robot_run_4legs_lib/Leg/Hip Actuator/Actuator/Controller ==
  K=bw*J/N : fl_lib/Physical Signals/Functions/PS Gain  gain=bw*J/N (N*m)/rad
  PS Add : fl_lib/Physical Signals/Functions/PS Add
  PS Add1 : fl_lib/Physical Signals/Functions/PS Add
  PS Gain : fl_lib/Physical Signals/Functions/PS Gain  gain=0.1 s
  r : PMIOPort  Side=Left
  w : PMIOPort  Port=2  Side=Left
  T : PMIOPort  Port=3  Side=Right
  q : PMIOPort  Port=4  Side=Left
  connections:
  PS Add1/LConn1 -- r/RConn1
  q/RConn1 -- PS Add/LConn2
  PS Add1/LConn2 -- PS Add/RConn1
  PS Gain/RConn1 -- PS Add/LConn1
  T/RConn1 -- K=bw*J/N/RConn1
  PS Add1/RConn1 -- K=bw*J/N/LConn1
  w/RConn1 -- PS Gain/LConn1
